simulink model "turbine"  (R2018a)
settings: Solver=VariableStepAuto  StartTime=0.0  StopTime=10  RelTol=1e-3
InitFcn:
  | init
values from neighbouring files (symbols this model uses):
  denGa = cell2mat(denGa)    [NikRaftar.m]    (also in main.m)
  denGb = cell2mat(denGb)    [NikRaftar.m]    (also in main.m)
  denGc = cell2mat(denGc)    [NikRaftar.m]    (also in main.m)
  denGd = cell2mat(denGd)    [NikRaftar.m]    (also in main.m)
  denGe = cell2mat(denGe)    [NikRaftar.m]    (also in main.m)
  denGf = cell2mat(denGf)    [NikRaftar.m]    (also in main.m)
  Kd_igv = .05    (= 0.05)    [NikRaftar.m]    (also in main.m)
  Kd_pd = .04    (= 0.04)    [NikRaftar.m]    (also in main.m)
  Ki_igv = .02    (= 0.02)    [NikRaftar.m]    (also in main.m)
  Ki_pd = .03    (= 0.03)    [NikRaftar.m]    (also in main.m)
  Kp_igv = 1    [NikRaftar.m]    (also in main.m)
  Kp_pd = 1    [NikRaftar.m]    (also in main.m)
  NoiseF = 0    [NikRaftar.m]    (also in main.m)
  NoiseIGV = 0    [NikRaftar.m]    (also in main.m)
  numGa = cell2mat(numGa)    [NikRaftar.m]    (also in main.m)
  numGb = cell2mat(numGb)    [NikRaftar.m]    (also in main.m)
  numGc = cell2mat(numGc)    [NikRaftar.m]    (also in main.m)
  numGd = cell2mat(numGd)    [NikRaftar.m]    (also in main.m)
  numGe = cell2mat(numGe)    [NikRaftar.m]    (also in main.m)
  numGf = cell2mat(numGf)    [NikRaftar.m]    (also in main.m)
libraries: simulink x6
settings Model: Creator=Mojtaba  LastModifiedBy=Mojtaba

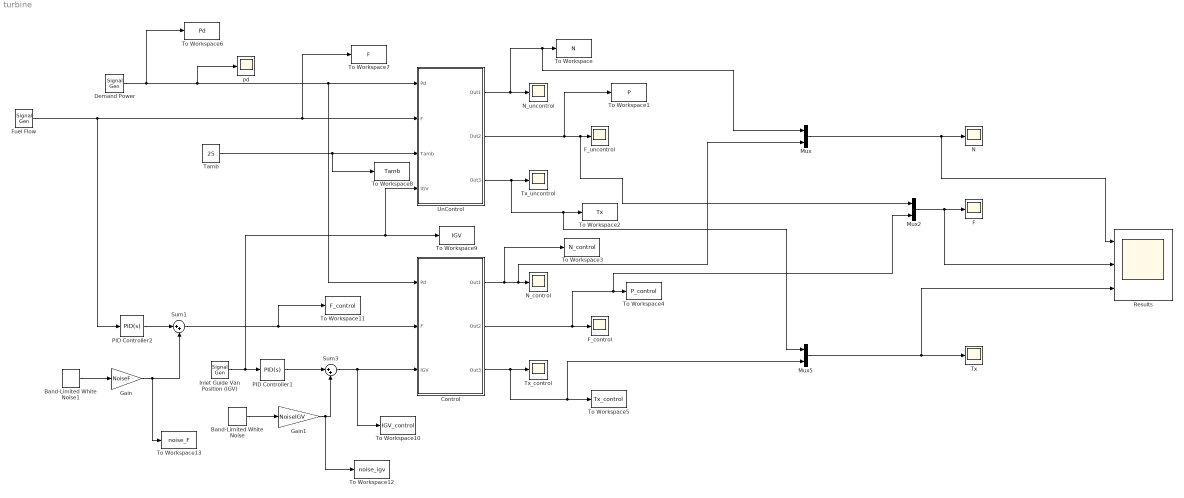
== system turbine ==
  Band-Limited White Noise : simulink/Sources/Band-Limited White Noise  Cov=[0.1]  Ts=0.1  seed=[23341]
  Band-Limited White Noise1 : simulink/Sources/Band-Limited White Noise  Cov=[0.1]  Ts=0.1  seed=[23341]
  "Control " : Subsystem
  Demand Power : SignalGenerator
  "F " : Scope
  F_control : Scope
  F_uncontrol : Scope
  "Fuel Flow " : SignalGenerator
  Gain : Gain  Gain=NoiseF
  Gain1 : Gain  Gain=NoiseIGV
  Inlet Guide Van Position (IGV) : SignalGenerator
  Mux : Mux  Inputs=2
  Mux2 : Mux  Inputs=2
  Mux5 : Mux  Inputs=2
  "N " : Scope
  N_control : Scope
  N_uncontrol : Scope
  PID Controller1 : simulink/Continuous/PID Controller  Controller=PID  TimeDomain=Continuous-time  SampleTime=-1  IntegratorMethod=Forward Euler  FilterMethod=Forward Euler  Form=Parallel  UseFilter=on  ControllerParametersSource=internal  P=Kp_igv  I=Ki_igv  D=Kd_igv  N=100  InitialConditionSource=internal  InitialConditionForIntegrator=0  InitialConditionForFilter=0  ExternalReset=none  LimitOutput=off  UpperSaturationLimit=inf  LowerSaturationLimit=-inf  LinearizeAsGain=on  AntiWindupMode=none  Kb=1  TrackingMode=off  Kt=1  PParamMin=[]  PParamMax=[]  IParamMin=[]  IParamMax=[]  DParamMin=[]  DParamMax=[]  NParamMin=[]  NParamMax=[]  KbParamMin=[]  KbParamMax=[]  KtParamMin=[]  KtParamMax=[]  POutMin=[]  POutMax=[]  IOutMin=[]  IOutMax=[]  DOutMin=[]  DOutMax=[]  NOutMin=[]  NOutMax=[]  KbOutMin=[]  KbOutMax=[]  KtOutMin=[]  KtOutMax=[]  IntegratorOutMin=[]  IntegratorOutMax=[]  FilterOutMin=[]  FilterOutMax=[]  SumOutMin=[]  SumOutMax=[]  SumI1OutMin=[]  SumI1OutMax=[]  SumI2OutMin=[]  SumI2OutMax=[]  SumI3OutMin=[]  SumI3OutMax=[]  SumDOutMin=[]  SumDOutMax=[]  SaturationOutMin=[]  SaturationOutMax=[]  IntegratorContinuousStateAttributes=''  IntegratorStateMustResolveToSignalObject=off  IntegratorRTWStateStorageClass=Auto  FilterContinuousStateAttributes=''  FilterStateMustResolveToSignalObject=off  FilterRTWStateStorageClass=Auto  DifferentiatorICPrevScaledInput=0  DifferentiatorOutMin=[]  DifferentiatorOutMax=[]  FilterDiffOutCoefMin=[]  FilterDiffOutCoefMax=[]  SumDenOutMin=[]  SumDenOutMax=[]  SumNumOutMin=[]  SumNumOutMax=[]  ReciprocalOutMin=[]  ReciprocalOutMax=[]  DivideOutMin=[]  DivideOutMax=[]  TunerSelectOption=Transfer Function Based (PID Tuner App)
  PID Controller2 : simulink/Continuous/PID Controller  Controller=PID  TimeDomain=Continuous-time  SampleTime=-1  IntegratorMethod=Forward Euler  FilterMethod=Forward Euler  Form=Parallel  UseFilter=on  ControllerParametersSource=internal  P=Kp_pd  I=Ki_pd  D=Kd_pd  N=100  InitialConditionSource=internal  InitialConditionForIntegrator=0  InitialConditionForFilter=0  ExternalReset=none  LimitOutput=off  UpperSaturationLimit=inf  LowerSaturationLimit=-inf  LinearizeAsGain=on  AntiWindupMode=none  Kb=1  TrackingMode=off  Kt=1  PParamMin=[]  PParamMax=[]  IParamMin=[]  IParamMax=[]  DParamMin=[]  DParamMax=[]  NParamMin=[]  NParamMax=[]  KbParamMin=[]  KbParamMax=[]  KtParamMin=[]  KtParamMax=[]  POutMin=[]  POutMax=[]  IOutMin=[]  IOutMax=[]  DOutMin=[]  DOutMax=[]  NOutMin=[]  NOutMax=[]  KbOutMin=[]  KbOutMax=[]  KtOutMin=[]  KtOutMax=[]  IntegratorOutMin=[]  IntegratorOutMax=[]  FilterOutMin=[]  FilterOutMax=[]  SumOutMin=[]  SumOutMax=[]  SumI1OutMin=[]  SumI1OutMax=[]  SumI2OutMin=[]  SumI2OutMax=[]  SumI3OutMin=[]  SumI3OutMax=[]  SumDOutMin=[]  SumDOutMax=[]  SaturationOutMin=[]  SaturationOutMax=[]  IntegratorContinuousStateAttributes=''  IntegratorStateMustResolveToSignalObject=off  IntegratorRTWStateStorageClass=Auto  FilterContinuousStateAttributes=''  FilterStateMustResolveToSignalObject=off  FilterRTWStateStorageClass=Auto  DifferentiatorICPrevScaledInput=0  DifferentiatorOutMin=[]  DifferentiatorOutMax=[]  FilterDiffOutCoefMin=[]  FilterDiffOutCoefMax=[]  SumDenOutMin=[]  SumDenOutMax=[]  SumNumOutMin=[]  SumNumOutMax=[]  ReciprocalOutMin=[]  ReciprocalOutMax=[]  DivideOutMin=[]  DivideOutMax=[]  TunerSelectOption=Transfer Function Based (PID Tuner App)
  "Results " : Scope  NumInputPorts=3
  Sum1 : Sum  Inputs=|++
  Sum3 : Sum  Inputs=|++
  Tamb : Constant  Value=25
  To Workspace : ToWorkspace  VariableName=N  SaveFormat=Timeseries  SampleTime=-1
  To Workspace1 : ToWorkspace  VariableName=P  SaveFormat=Timeseries  SampleTime=-1
  To Workspace10 : ToWorkspace  VariableName=IGV_control  SaveFormat=Timeseries  SampleTime=-1
  To Workspace11 : ToWorkspace  VariableName=F_control  SaveFormat=Timeseries  SampleTime=-1
  To Workspace12 : ToWorkspace  VariableName=noise_igv  SaveFormat=Timeseries  SampleTime=-1
  To Workspace13 : ToWorkspace  VariableName=noise_F  SaveFormat=Timeseries  SampleTime=-1
  To Workspace2 : ToWorkspace  VariableName=Tx  SaveFormat=Timeseries  SampleTime=-1
  To Workspace3 : ToWorkspace  VariableName=N_control  SaveFormat=Timeseries  SampleTime=-1
  To Workspace4 : ToWorkspace  VariableName=P_control  SaveFormat=Timeseries  SampleTime=-1
  To Workspace5 : ToWorkspace  VariableName=Tx_control  SaveFormat=Timeseries  SampleTime=-1
  To Workspace6 : ToWorkspace  VariableName=Pd  SaveFormat=Timeseries  SampleTime=-1
  To Workspace7 : ToWorkspace  VariableName=F  SaveFormat=Timeseries  SampleTime=-1
  To Workspace8 : ToWorkspace  VariableName=Tamb  SaveFormat=Timeseries  SampleTime=-1
  To Workspace9 : ToWorkspace  VariableName=IGV  SaveFormat=Timeseries  SampleTime=-1
  "Tx " : Scope
  "Tx_control " : Scope
  "Tx_uncontrol " : Scope
  UnControl : Subsystem
  "pd " : Scope
  wires:
  UnControl/1(Out1) -> Mux/1, To Workspace/1, N_uncontrol/1
  UnControl/2(Out2) -> To Workspace1/1, Mux2/1, F_uncontrol/1
  UnControl/3(Out3) -> Mux5/1, To Workspace2/1, "Tx_uncontrol "/1
  "Control "/3(Out3) -> Mux5/2, To Workspace5/1, "Tx_control "/1
  "Control "/2(Out2) -> Mux2/2, To Workspace4/1, F_control/1
  "Control "/1(Out1) -> To Workspace3/1, Mux/2, N_control/1
  "Fuel Flow "/1 -> PID Controller2/1, To Workspace7/1, UnControl/2(F)
  Tamb/1 -> UnControl/3(Tamb), To Workspace8/1
  Inlet Guide Van Position (IGV)/1 -> UnControl/4(IGV), To Workspace9/1, PID Controller1/1
  Demand Power/1 -> To Workspace6/1, "pd "/1, "Control "/1("Pd "), UnControl/1(Pd)
  Mux/1 -> "Results "/1, "N "/1
  Mux2/1 -> "Results "/2, "F "/1
  Mux5/1 -> "Results "/3, "Tx "/1
  Sum3/1 -> To Workspace10/1, "Control "/3("IGV ")
  Band-Limited White Noise/1 -> Gain1/1
  Sum1/1 -> To Workspace11/1, "Control "/2(F)
  Band-Limited White Noise1/1 -> Gain/1
  Gain/1 -> To Workspace13/1, Sum1/2
  PID Controller2/1 -> Sum1/1
  Gain1/1 -> To Workspace12/1, Sum3/2
  PID Controller1/1 -> Sum3/1

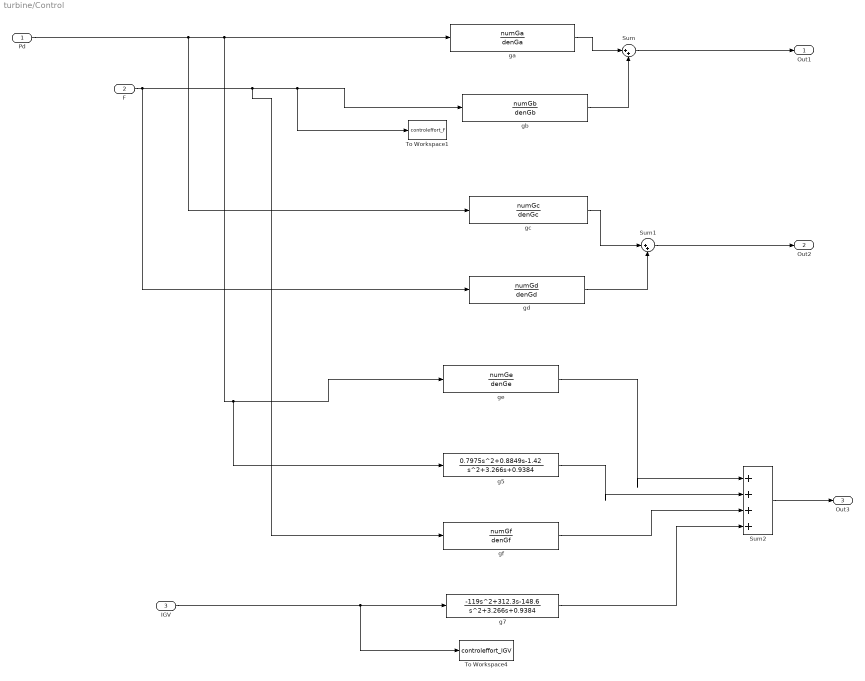
== system turbine/Control  ==
  "Pd " : Inport
  F : Inport  Port=2
  "IGV " : Inport  Port=3
  Sum : Sum  Inputs=|++
  Sum1 : Sum  Inputs=|++
  Sum2 : Sum  Inputs=|++++
  To Workspace1 : ToWorkspace  VariableName=controleffort_F  SaveFormat=Timeseries  SampleTime=-1
  To Workspace4 : ToWorkspace  VariableName=controleffort_IGV  SaveFormat=Timeseries  SampleTime=-1
  g5 : TransferFcn  Numerator=[0.7975,0.8849,-1.42]  Denominator=[1,3.266,0.9384]
  g7 : TransferFcn  Numerator=[-119,312.3,-148.6]  Denominator=[1,3.266,0.9384]
  "ga " : TransferFcn  Numerator=numGa  Denominator=denGa
  "gb " : TransferFcn  Numerator=numGb  Denominator=denGb
  gc : TransferFcn  Numerator=numGc  Denominator=denGc
  gd : TransferFcn  Numerator=numGd  Denominator=denGd
  ge : TransferFcn  Numerator=numGe  Denominator=denGe
  gf : TransferFcn  Numerator=numGf  Denominator=denGf
  Out1 : Outport
  Out2 : Outport  Port=2
  Out3 : Outport  Port=3
  wires:
  Sum/1 -> Out1/1
  Sum1/1 -> Out2/1
  Sum2/1 -> Out3/1
  gc/1 -> Sum1/1
  g5/1 -> Sum2/2
  gf/1 -> Sum2/3
  g7/1 -> Sum2/4
  ge/1 -> Sum2/1
  gd/1 -> Sum1/2
  "gb "/1 -> Sum/2
  "ga "/1 -> Sum/1
  "Pd "/1 -> gc/1, "ga "/1, ge/1, g5/1
  "IGV "/1 -> g7/1, To Workspace4/1
  F/1 -> gd/1, To Workspace1/1, "gb "/1, gf/1

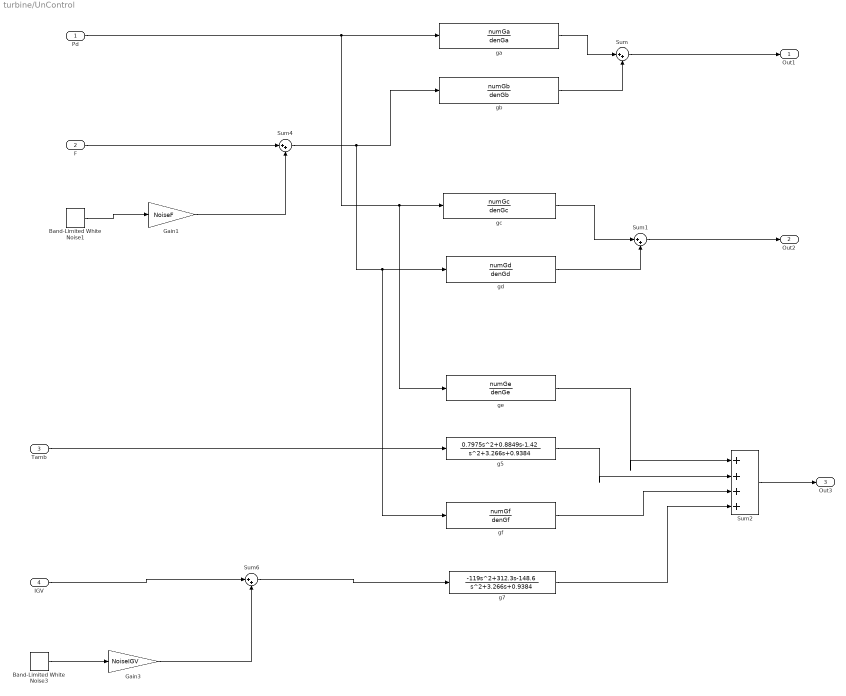
== system turbine/UnControl ==
  Pd : Inport
  F : Inport  Port=2
  Tamb : Inport  Port=3
  IGV : Inport  Port=4
  Band-Limited White Noise1 : simulink/Sources/Band-Limited White Noise  Cov=[0.1]  Ts=0.1  seed=[23341]
  Band-Limited White Noise3 : simulink/Sources/Band-Limited White Noise  Cov=[0.1]  Ts=0.1  seed=[23341]
  Gain1 : Gain  Gain=NoiseF
  Gain3 : Gain  Gain=NoiseIGV
  Sum{,1,4,6} (4 alike) : Sum  Inputs=|++
  Sum2 : Sum  Inputs=|++++
  g5 : TransferFcn  Numerator=[0.7975,0.8849,-1.42]  Denominator=[1,3.266,0.9384]
  g7 : TransferFcn  Numerator=[-119,312.3,-148.6]  Denominator=[1,3.266,0.9384]
  "ga " : TransferFcn  Numerator=numGa  Denominator=denGa
  "gb " : TransferFcn  Numerator=numGb  Denominator=denGb
  gc : TransferFcn  Numerator=numGc  Denominator=denGc
  gd : TransferFcn  Numerator=numGd  Denominator=denGd
  ge : TransferFcn  Numerator=numGe  Denominator=denGe
  gf : TransferFcn  Numerator=numGf  Denominator=denGf
  Out1 : Outport
  Out2 : Outport  Port=2
  Out3 : Outport  Port=3
  wires:
  "ga "/1 -> Sum/1
  "gb "/1 -> Sum/2
  gd/1 -> Sum1/2
  IGV/1 -> Sum6/1
  ge/1 -> Sum2/1
  g7/1 -> Sum2/4
  gf/1 -> Sum2/3
  g5/1 -> Sum2/2
  F/1 -> Sum4/1
  gc/1 -> Sum1/1
  Sum2/1 -> Out3/1
  Sum1/1 -> Out2/1
  Sum/1 -> Out1/1
  Pd/1 -> "ga "/1, ge/1, gc/1
  Band-Limited White Noise1/1 -> Gain1/1
  Gain1/1 -> Sum4/2
  Sum4/1 -> gf/1, gd/1, "gb "/1
  Tamb/1 -> g5/1
  Band-Limited White Noise3/1 -> Gain3/1
  Gain3/1 -> Sum6/2
  Sum6/1 -> g7/1
